simulink model "single_phase_afe_ttype"  (R2026b)
settings: Solver=ode23tb  StopTime=param.sim.simlength  FixedStep=param.sim.tc  MaxStep=param.glb_time.tc
values from neighbouring files (symbols this model uses):
  param = struct()    [init_model.m]
undefined symbols (not defined in the file or in its folder): magnitude
libraries: fl_lib x30, nesl_utility x22, single_phase_transformer_lib x3, phase_shift_filter_ccaller x2, lithium_ion_battery x1, dclink_for_three_levels x1, three_phase_voltage_with_frt_emulator x1, power_meter_iec x1, simulink x1, cstblocks_lti x1, single_phase_three_levels_PWM_modulator x1, moving_average_filter x1
(part 1 of 4)
settings Model: Creator=LTNBDA  LastModifiedBy=d.bagnara
settings SolverCC: AutoInsertRateTranBlk=on  SolverResetMethod=Robust  ZeroCrossAlgorithm=Adaptive  ZeroCrossControl=EnableAll
settings DataIOCC: DSMLogging=off  LimitDataPoints=on  MaxDataPoints=1  ReturnWorkspaceOutputs=off  SaveFormat=Array  SaveOutput=off  SaveTime=off  SignalLogging=off  SignalLoggingSaveFormat=ModelDataLogs
settings OptimizationCC: EfficientMapNaN2IntZero=off  LifeSpan=inf  MemsetInitFltsAndDblsToZero=off
settings DebuggingCC: ArithmeticOperatorsInVariantConditions=warning  FcnCallInpInsideContextMsg=warning  IgnoredZcDiagnostic=none  MergeDetectMultiDrivingBlocksExec=none  MultiTaskCondExecSysMsg=none  MultiTaskDSMMsg=warning  MultiTaskRateTransMsg=warning  SFNoUnconditionalDefaultTransitionDiag=warning  SFUnexpectedBacktrackingDiag=warning  SaveWithParameterizedLinksMsg=none  SignalResolutionControl=TryResolveAllWithWarning  SolverPrmCheckMsg=warning  StateNameClashWarn=warning  UnderspecifiedInitializationDetection=Classic
settings HardwareCC: ProdEndianess=Unspecified  ProdEqTarget=off  ProdHWDeviceType=Generic->64-bit Embedded Processor (LP64)  ProdIntDivRoundTo=Undefined  ProdLargestAtomicFloat=None  TargetEndianess=LittleEndian  TargetHWDeviceType=MATLAB Host  TargetIntDivRoundTo=Zero  TargetLongLongMode=on
settings ModelReferenceCC: PropagateSignalLabelsOutOfModel=off
settings SFSimCC: CustomCodeUndefinedFunction=UseInterfaceOnly  SimUseLocalCustomCode=off
settings SFSimCC: SimCustomHeaderCode=|
  | #include "rpi.h"
  | #include "rpi_simulink.h"
  | #include "mavgflt.h"
  | #include "mavgflt_simulink.h"
  | #include "mavgflts.h"
  | #include "mavgflts_simulink.h"
  | #include "dsmavgflt.h"
  | #include "dsmavgflt_simulink.h"
  | #include "bemf_obsv.h"
  | #include "bemf_obsv_simulink.h"
  | #include "bemf_obsv_load_est.h"
  | #include "bemf_obsv_load_est_simulink.h"
  | #include "dqvector_pi.h"
  | #include "dqvector_pi_simulink.h"
  | #include "sv_pwm_simulink.h"
  | #include "sv_pwm.h"
  | #include "first_harmonic_tracker.h"
  | #include "first_harmonic_tracker_simulink.h"
  | #include "dqpll_thyr.h"
  | #include "dqpll_thyr_simulink.h"
  | #include "dqpll_grid.h"
  | #include "dqpll_grid_simulink.h"
  | #include "phase_shift_flt_simulink.h"
  | #include "phase_shift_flt.h"
  | #include "sogi_flt_simulink.h"
  | #include "sogi_flt.h"
  | #include "linear_double_integrator_observer_simulink.h"
  | #include "linear_double_integrator_observer.h"
settings SFSimCC: SimUserIncludeDirs=|
  | include
  | src
settings SFSimCC: SimUserSources=|
  | "rpi.c"
  | "rpi_simulink.c"
  | "mavgflt_simulink.c"
  | "mavgflt.c"
  | "mavgflts_simulink.c"
  | "mavgflts.c"
  | "dsmavgflt_simulink.c"
  | "dsmavgflt.c"
  | "bemf_obsv_simulink.c"
  | "bemf_obsv.c"
  | "bemf_obsv_load_est_simulink.c"
  | "bemf_obsv_load_est.c"
  | "dqvector_pi.c"
  | "dqvector_pi_simulink.c"
  | "sv_pwm_simulink.c"
  | "sv_pwm.c"
  | "first_harmonic_tracker_simulink.c"
  | "first_harmonic_tracker.c"
  | "dqpll_thyr_simulink.c"
  | "dqpll_thyr.c"
  | "dqpll_grid_simulink.c"
  | "dqpll_grid.c"
  | "phase_shift_flt_simulink.c"
  | "phase_shift_flt.c"
  | "sogi_flt_simulink.c"
  | "sogi_flt.c"
  | "linear_double_integrator_observer_simulink.c"
  | "linear_double_integrator_observer.c"
settings RTWCC: RTWUseLocalCustomCode=off
settings CodeAppCC: StateflowObjectComments=on
settings GRTTargetCC: CombineOutputUpdateFcns=off  GRTInterface=on  TargetLangStandard=C89/C90 (ANSI)
settings ConfigComp: CovExternalEMLEnable=off  CovSaveCumulativeToWorkspaceVar=on  CovSaveSingleToWorkspaceVar=on
settings SimscapeCC: SimscapeNormalizeSystem=off  SimscapeUseEnergyAccounting=off

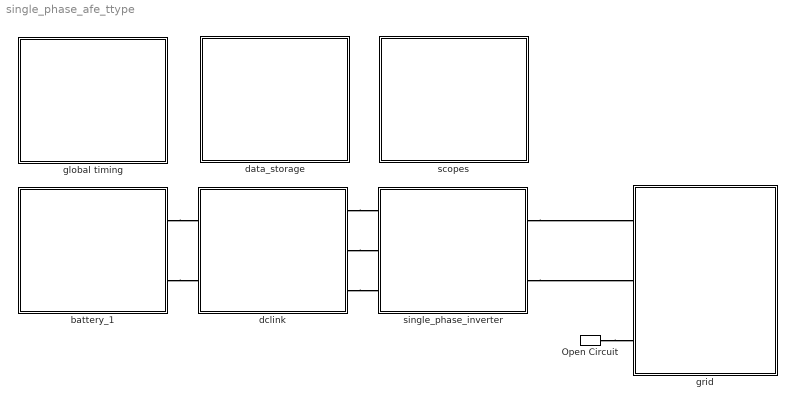
== system single_phase_afe_ttype ==
  Open Circuit : fl_lib/Electrical/Electrical Elements/Open Circuit  v_specify=off  v_priority=None  v=0 V  v_nominal_specify=off  v_nominal_value=1  v_nominal_unit=V
  battery_1 : Subsystem
  data_storage : Subsystem
  dclink : Subsystem
  global timing : Subsystem
  grid : Subsystem
  scopes : Subsystem
  single_phase_inverter : Subsystem
  connections:
  single_phase_inverter/RConn1 -- grid/RConn1
  single_phase_inverter/RConn2 -- grid/RConn2
  dclink/RConn1 -- single_phase_inverter/LConn1
  dclink/RConn2 -- single_phase_inverter/LConn2
  dclink/RConn3 -- single_phase_inverter/LConn3
  battery_1/RConn2 -- dclink/LConn2
  battery_1/RConn1 -- dclink/LConn1
  Open Circuit/LConn1 -- grid/RConn3

== system single_phase_afe_ttype/battery_1 ==
  To Workspace14 : ToWorkspace  VariableName=battery_1_data_sim  SampleTime=param.glb_time.tc
      settings: MaxDataPoints=param.glb_time.Nc  Decimation=param.glb_time.decimation_tc
  lithium ion battery : Scope
      settings: ActiveDisplayYMinimum=-1009.2320386548216  ActiveDisplayYMaximum=1611.8768779635091  DataLoggingVariableName=ScopeData3
  lithium_ion_battery : lithium_ion_battery/lithium_ion_battery  Q=param.battery.pack_1.Q  number_of_cells=param.battery.pack_1.number_of_cells  E_1=param.battery.pack_1.E_1  E0=param.battery.pack_1.E0  E1=param.battery.pack_1.E1  E2=param.battery.pack_1.E2  E3=param.battery.pack_1.E3  Elog=param.battery.pack_1.Elog  R0=param.battery.pack_1.R0  R1=param.battery.pack_1.R1  C1=param.battery.pack_1.C1  M=param.battery.pack_1.M  alpha=param.battery.pack_1.alpha  soc_init=param.battery.pack_1.soc_init  ts_battery=param.glb_time.ts_dab  q1Kalman=param.battery.pack_1.q1Kalman  q2Kalman=param.battery.pack_1.q2Kalman  q3Kalman=param.battery.pack_1.q3Kalman  rKalman=param.battery.pack_1.rKalman  tc=param.glb_time.tc  enable_white_noise_m=0  battery_voltage_init_m=param.battery.nominal_battery_voltage_1
  single_phase_ui_measure : Subsystem
  dc(+) : PMIOPort  Side=Right
  dc(-) : PMIOPort  Port=2  Side=Right
  wires:
  lithium_ion_battery/1 -> To Workspace14/1, lithium ion battery/1
  connections:
  single_phase_ui_measure/LConn2 -- lithium_ion_battery/RConn2
  single_phase_ui_measure/RConn1 -- dc(+)/RConn1
  single_phase_ui_measure/LConn1 -- lithium_ion_battery/RConn1
  dc(-)/RConn1 -- single_phase_ui_measure/RConn2

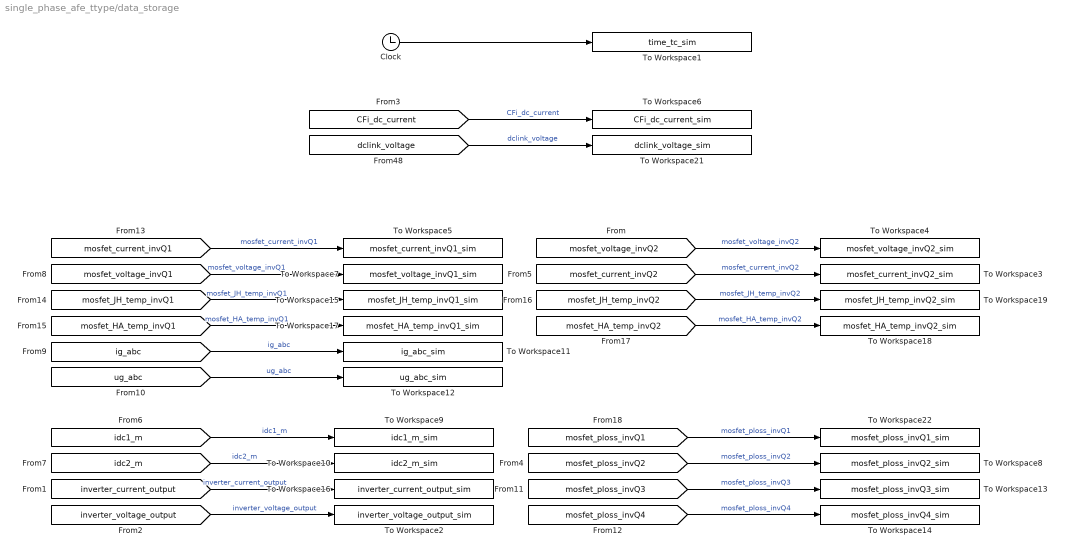
== system single_phase_afe_ttype/data_storage ==
  Clock : Clock
  To Workspace1 : ToWorkspace  VariableName=time_tc_sim  SampleTime=param.glb_time.tc
      settings: MaxDataPoints=param.glb_time.Nc  Decimation=param.glb_time.decimation_tc
  To Workspace10 : ToWorkspace  VariableName=idc2_m_sim  SampleTime=param.glb_time.tc
      settings: MaxDataPoints=param.glb_time.Nc  Decimation=param.glb_time.decimation_tc
  To Workspace11 : ToWorkspace  VariableName=ig_abc_sim  SampleTime=param.glb_time.tc
      settings: MaxDataPoints=param.glb_time.Nc  Decimation=param.glb_time.decimation_tc
  To Workspace12 : ToWorkspace  VariableName=ug_abc_sim  SampleTime=param.glb_time.tc
      settings: MaxDataPoints=param.glb_time.Nc  Decimation=param.glb_time.decimation_tc
  To Workspace13 : ToWorkspace  VariableName=mosfet_ploss_invQ3_sim  SampleTime=param.glb_time.tc
      settings: MaxDataPoints=param.glb_time.Nc  Decimation=param.glb_time.decimation_tc
  To Workspace14 : ToWorkspace  VariableName=mosfet_ploss_invQ4_sim  SampleTime=param.glb_time.tc
      settings: MaxDataPoints=param.glb_time.Nc  Decimation=param.glb_time.decimation_tc
  To Workspace15 : ToWorkspace  VariableName=mosfet_JH_temp_invQ1_sim  SampleTime=param.glb_time.tc
      settings: MaxDataPoints=param.glb_time.Nc  Decimation=param.glb_time.decimation_tc
  To Workspace16 : ToWorkspace  VariableName=inverter_current_output_sim  SampleTime=param.glb_time.tc
      settings: MaxDataPoints=param.glb_time.Nc  Decimation=param.glb_time.decimation_tc
  To Workspace17 : ToWorkspace  VariableName=mosfet_HA_temp_invQ1_sim  SampleTime=param.glb_time.tc
      settings: MaxDataPoints=param.glb_time.Nc  Decimation=param.glb_time.decimation_tc
  To Workspace18 : ToWorkspace  VariableName=mosfet_HA_temp_invQ2_sim  SampleTime=param.glb_time.tc
      settings: MaxDataPoints=param.glb_time.Nc  Decimation=param.glb_time.decimation_tc
  To Workspace19 : ToWorkspace  VariableName=mosfet_JH_temp_invQ2_sim  SampleTime=param.glb_time.tc
      settings: MaxDataPoints=param.glb_time.Nc  Decimation=param.glb_time.decimation_tc
  To Workspace2 : ToWorkspace  VariableName=inverter_voltage_output_sim  SampleTime=param.glb_time.tc
      settings: MaxDataPoints=param.glb_time.Nc  Decimation=param.glb_time.decimation_tc
  To Workspace21 : ToWorkspace  VariableName=dclink_voltage_sim  SampleTime=param.glb_time.tc
      settings: MaxDataPoints=param.glb_time.Nc  Decimation=param.glb_time.decimation_tc
  To Workspace22 : ToWorkspace  VariableName=mosfet_ploss_invQ1_sim  SampleTime=param.glb_time.tc
      settings: MaxDataPoints=param.glb_time.Nc  Decimation=param.glb_time.decimation_tc
  To Workspace3 : ToWorkspace  VariableName=mosfet_current_invQ2_sim  SampleTime=param.glb_time.tc
      settings: MaxDataPoints=param.glb_time.Nc  Decimation=param.glb_time.decimation_tc
  To Workspace4 : ToWorkspace  VariableName=mosfet_voltage_invQ2_sim  SampleTime=param.glb_time.tc
      settings: MaxDataPoints=param.glb_time.Nc  Decimation=param.glb_time.decimation_tc
  To Workspace5 : ToWorkspace  VariableName=mosfet_current_invQ1_sim  SampleTime=param.glb_time.tc
      settings: MaxDataPoints=param.glb_time.Nc  Decimation=param.glb_time.decimation_tc
  To Workspace6 : ToWorkspace  VariableName=CFi_dc_current_sim  SampleTime=param.glb_time.tc
      settings: MaxDataPoints=param.glb_time.Nc  Decimation=param.glb_time.decimation_tc
  To Workspace7 : ToWorkspace  VariableName=mosfet_voltage_invQ1_sim  SampleTime=param.glb_time.tc
      settings: MaxDataPoints=param.glb_time.Nc  Decimation=param.glb_time.decimation_tc
  To Workspace8 : ToWorkspace  VariableName=mosfet_ploss_invQ2_sim  SampleTime=param.glb_time.tc
      settings: MaxDataPoints=param.glb_time.Nc  Decimation=param.glb_time.decimation_tc
  To Workspace9 : ToWorkspace  VariableName=idc1_m_sim  SampleTime=param.glb_time.tc
      settings: MaxDataPoints=param.glb_time.Nc  Decimation=param.glb_time.decimation_tc
  wires:
  Clock/1 -> To Workspace1/1
  [inverter_current_output] -> To Workspace16/1  "inverter_current_output"
  [inverter_voltage_output] -> To Workspace2/1  "inverter_voltage_output"
  [CFi_dc_current] -> To Workspace6/1  "CFi_dc_current"
  [mosfet_ploss_invQ1] -> To Workspace22/1  "mosfet_ploss_invQ1"
  [dclink_voltage] -> To Workspace21/1  "dclink_voltage"
  [mosfet_current_invQ1] -> To Workspace5/1  "mosfet_current_invQ1"
  [mosfet_current_invQ2] -> To Workspace3/1  "mosfet_current_invQ2"
  [mosfet_voltage_invQ2] -> To Workspace4/1  "mosfet_voltage_invQ2"
  [mosfet_voltage_invQ1] -> To Workspace7/1  "mosfet_voltage_invQ1"
  [mosfet_ploss_invQ2] -> To Workspace8/1  "mosfet_ploss_invQ2"
  [ig_abc] -> To Workspace11/1  "ig_abc"
  [ug_abc] -> To Workspace12/1  "ug_abc"
  [mosfet_JH_temp_invQ1] -> To Workspace15/1  "mosfet_JH_temp_invQ1"
  [mosfet_HA_temp_invQ1] -> To Workspace17/1  "mosfet_HA_temp_invQ1"
  [mosfet_JH_temp_invQ2] -> To Workspace19/1  "mosfet_JH_temp_invQ2"
  [mosfet_HA_temp_invQ2] -> To Workspace18/1  "mosfet_HA_temp_invQ2"
  [idc1_m] -> To Workspace9/1  "idc1_m"
  [idc2_m] -> To Workspace10/1  "idc2_m"
  [mosfet_ploss_invQ4] -> To Workspace14/1  "mosfet_ploss_invQ4"
  [mosfet_ploss_invQ3] -> To Workspace13/1  "mosfet_ploss_invQ3"

== system single_phase_afe_ttype/dclink ==
  Open Circuit : fl_lib/Electrical/Electrical Elements/Open Circuit  v_specify=off  v_priority=None  v=0 V  v_nominal_specify=off  v_nominal_value=1  v_nominal_unit=V
  dclink : dclink_for_three_levels/dclink  Cdc1_m=param.afe.hw.CFi1  Cdc2_m=param.afe.hw.CFi2  Rudc_measure=param.afe.hw.Rudc_measure  Vdc_scale=param.afe.hw.udc_nom  Vdc1_m_init=param.afe.hw.udc1_init  Vdc2_m_init=param.afe.hw.udc2_init
  references : Subsystem
  Udc(+) : PMIOPort  Side=Right
  np : PMIOPort  Port=2  Side=Right
  Udc(-) : PMIOPort  Port=3  Side=Right
  udc(+) : PMIOPort  Port=4  Side=Left
  udc(-) : PMIOPort  Port=5  Side=Left
  wires:
  dclink/1 -> references/1(m)
  connections:
  Open Circuit/LConn1 -- dclink/RConn2
  udc(+)/RConn1 -- dclink/RConn1
  udc(-)/RConn1 -- dclink/RConn3
  Udc(+)/RConn1 -- dclink/LConn1
  Udc(-)/RConn1 -- dclink/LConn3
  dclink/LConn2 -- np/RConn1

== system single_phase_afe_ttype/global timing ==
  Unit Delay : UnitDelay  SampleTime=param.glb_time.tc
  time_afe1 : Subsystem  mask{k=1}
      mask prompts: k "Time Gain"
      mask Display:
      | disp('time-gen');
      | port_label('input', 1, 'crt');
      | port_label('output', 1, 'tout');
  time_afe3 : Subsystem  mask{k=1}
      mask prompts: k "Time Gain"
      mask Display:
      | disp('time-gen');
      | port_label('output', 1, 'tout');
  tag scope: master_time=global, time_inv_module_1=global
  wires:
  time_afe1/1(Out1) -> [time_inv_module_1]
  time_afe3/1(Out1) -> [master_time]
  [local_time_corr_llc_mod1] -> Unit Delay/1
  Unit Delay/1 -> time_afe1/1(correction_time)

== system single_phase_afe_ttype/grid ==
  Bus Selector : BusSelector  OutputSignals=Q1p,Q1n,P1n,P1p,U1n,U1p,i_act_1n,i_react_1n,i_act_1p,i_react_1p
  To Workspace1 : ToWorkspace  VariableName=i_react_1n  SampleTime=param.glb_time.ts_afe
      settings: MaxDataPoints=param.glb_time.Ns_afe
  To Workspace2 : ToWorkspace  VariableName=i_react_1p  SampleTime=param.glb_time.ts_afe
      settings: MaxDataPoints=param.glb_time.Ns_afe
  To Workspace3 : ToWorkspace  VariableName=i_act_1n  SampleTime=param.glb_time.ts_afe
      settings: MaxDataPoints=param.glb_time.Ns_afe
  To Workspace4 : ToWorkspace  VariableName=i_act_1p  SampleTime=param.glb_time.ts_afe
      settings: MaxDataPoints=param.glb_time.Ns_afe
  To Workspace5 : ToWorkspace  VariableName=u1p  SampleTime=param.glb_time.ts_afe
      settings: MaxDataPoints=param.glb_time.Ns_afe
  To Workspace6 : ToWorkspace  VariableName=u1n  SampleTime=param.glb_time.ts_afe
      settings: MaxDataPoints=param.glb_time.Ns_afe
  grid_emulator : Subsystem
  power meter iec1 : power_meter_iec/power meter iec  period=pi/param.grid.emu.omega_grid_nom  ts=param.glb_time.tc  enable_time=0.025
  threephase_vi_measures : Subsystem
  ua : PMIOPort  Side=Right
  ub : PMIOPort  Port=2  Side=Right
  uc : PMIOPort  Port=3  Side=Right
  tag scope: P1n_global=global, P1p_global=global, Q1n_global=global, Q1p_global=global
  wires:
  [gamma_grid_emulator] -> power meter iec1/1
  [ug_abc] -> power meter iec1/2
  [ig_abc] -> power meter iec1/3
  power meter iec1/1 -> Bus Selector/1
  Bus Selector/1 -> [Q1p_global]  "<Q1p>"
  Bus Selector/2 -> [Q1n_global]  "<Q1n>"
  Bus Selector/3 -> [P1n_global]  "<P1n>"
  Bus Selector/4 -> [P1p_global]  "<P1p>"
  Bus Selector/5 -> To Workspace6/1  "<U1n>"
  Bus Selector/6 -> To Workspace5/1  "<U1p>"
  Bus Selector/7 -> To Workspace3/1  "<i_act_1n>"
  Bus Selector/8 -> To Workspace1/1  "<i_react_1n>"
  Bus Selector/9 -> To Workspace4/1  "<i_act_1p>"
  Bus Selector/10 -> To Workspace2/1  "<i_react_1p>"
  [omega_grid_emulator] -> power meter iec1/4
  connections:
  threephase_vi_measures/LConn3 -- grid_emulator/RConn3
  threephase_vi_measures/LConn1 -- grid_emulator/RConn1
  threephase_vi_measures/RConn2 -- ub/RConn1
  threephase_vi_measures/LConn2 -- grid_emulator/RConn2
  threephase_vi_measures/RConn1 -- ua/RConn1
  threephase_vi_measures/RConn3 -- uc/RConn1

== system single_phase_afe_ttype/scopes ==
  Bus Creator : BusCreator  Inputs=2
  dclink voltage : Scope  NumInputPorts=3
      settings: SampleTime=param.glb_time.tc  ActiveDisplayString=3  ActiveDisplayYMinimum=-1788.34839052713  ActiveDisplayYMaximum=517.01346635999766  DataLoggingVariableName=ScopeData9
  ig_abc/ug_abc : Scope  NumInputPorts=2
      settings: SampleTime=param.glb_time.tc  ActiveDisplayYMinimum=-713.27946799108952  ActiveDisplayYMaximum=713.52801996826327  DataLoggingVariableName=ScopeData5
  input dc modA : Scope  NumInputPorts=2
      settings: SampleTime=param.glb_time.tc  ActiveDisplayYMinimum=-67.715483087935809  ActiveDisplayYMaximum=609.43655738592645  DataLoggingVariableName=ScopeData4
  inverter current/voltage : Scope  NumInputPorts=4
      settings: ActiveDisplayString=3  ActiveDisplayYMinimum=-1356.3487617019355  ActiveDisplayYMaximum=1011.5095624681422
  inverter current/voltage output : Scope  NumInputPorts=2
      settings: ActiveDisplayYMinimum=-809.40125502350236  ActiveDisplayYMaximum=818.72199299199281
  iu-mosfet-invQ1 : Scope  NumInputPorts=2
      settings: SampleTime=param.glb_time.tc  ActiveDisplayYMinimum=-1884.5917198054758  ActiveDisplayYMaximum=2532.7760155502147  DataLoggingVariableName=ScopeData7
  power_loss mosfet_inv : Scope  NumInputPorts=2
      settings: SampleTime=param.glb_time.tc  ActiveDisplayYMinimum=-70.3597503046535  ActiveDisplayYMaximum=633.23512274412  DataLoggingVariableName=ScopeData6
  wires:
  [idc1_m] -> inverter current/voltage/3  "idc1_m"
  [inverter_voltage_output] -> inverter current/voltage/2, inverter current/voltage output/1  "inverter_voltage_output_modA"
  [inverter_current_output] -> inverter current/voltage/1, inverter current/voltage output/2  "inverter_current_output_modA"
  [idc2_m] -> inverter current/voltage/4  "idc2_m"
  [idc1_m] -> input dc modA/1  "idc1_m"
  [idc2_m] -> input dc modA/2  "idc2_m"
  [ug_abc] -> ig_abc/ug_abc/2  "vg_abc"
  [ig_abc] -> ig_abc/ug_abc/1  "ig_abc"
  [mosfet_ploss_invQ1] -> power_loss mosfet_inv/1  "mosfet_ploss_invQ1"
  [mosfet_JH_temp_invQ1] -> Bus Creator/1  "mosfet_JH_temp_invQ1"
  [mosfet_HA_temp_invQ1] -> Bus Creator/2  "mosfet_HA_temp_invQ1"
  Bus Creator/1 -> power_loss mosfet_inv/2
  [mosfet_current_invQ1] -> iu-mosfet-invQ1/1  "mosfet_current_invQ1"
  [mosfet_voltage_invQ1] -> iu-mosfet-invQ1/2  "mosfet_voltage_invQ1"
  [dclink_voltage] -> dclink voltage/1  "dclink_voltage"
  [dclink_p2gnd_voltage] -> dclink voltage/2  "dclink_p2gnd_voltage"
  [dclink_n2gnd_voltage] -> dclink voltage/3  "dclink_n2gnd_voltage"

== system single_phase_afe_ttype/single_phase_inverter ==
  CFu : fl_lib/Electrical/Electrical Elements/Capacitor  c=param.afe.hw.CFu F  r=param.afe.hw.RCFu Ohm  g=0 1/Ohm  i_specify=off  i_priority=None  i=0 A  i_nominal_specify=off  i_nominal_value=1  i_nominal_unit=A  v_specify=off  v_priority=None  v=0 V  v_nominal_specify=off  v_nominal_value=1  v_nominal_unit=V  vc_specify=off  vc_priority=High  vc=0 V  vc_nominal_specify=off  vc_nominal_value=1  vc_nominal_unit=V
  LFu1 : fl_lib/Electrical/Electrical Elements/Inductor  l=param.afe.hw.LFu1 H  r=param.afe.hw.RLFu1 Ohm  g=1e-9 1/Ohm  i_specify=on  i_priority=High  i=0 A  i_nominal_specify=off  i_nominal_value=1  i_nominal_unit=A  v_specify=off  v_priority=None  v=0 V  v_nominal_specify=off  v_nominal_value=1  v_nominal_unit=V  i_L_specify=off  i_L_priority=High  i_L=0 A  i_L_nominal_specify=off  i_L_nominal_value=1  i_L_nominal_unit=A
  LFu2 : fl_lib/Electrical/Electrical Elements/Inductor  l=param.afe.hw.LFu2 H  r=param.afe.hw.RLFu2 Ohm  g=1e-9 1/Ohm  i_specify=on  i_priority=High  i=0 A  i_nominal_specify=off  i_nominal_value=1  i_nominal_unit=A  v_specify=off  v_priority=None  v=0 V  v_nominal_specify=off  v_nominal_value=1  v_nominal_unit=V  i_L_specify=off  i_L_priority=High  i_L=0 A  i_L_nominal_specify=off  i_L_nominal_value=1  i_L_nominal_unit=A
  single phase inverter control : Subsystem
  single_phase_inverter : Subsystem
  vi_measures_grid : Subsystem
  uac(+) : PMIOPort  Side=Right
  uac(-) : PMIOPort  Port=2  Side=Right
  udc(+) : PMIOPort  Port=3  Side=Left
  np : PMIOPort  Port=4  Side=Left
  udc(-) : PMIOPort  Port=5  Side=Left
  wires:
  single phase inverter control/1(gate_cmds) -> single_phase_inverter/1(gate_commands)
  connections:
  single_phase_inverter/LConn1 -- udc(+)/RConn1
  np/RConn1 -- single_phase_inverter/LConn2
  single_phase_inverter/LConn3 -- udc(-)/RConn1
  LFu1/RConn1 -- vi_measures_grid/RConn1 -- CFu/LConn1
  LFu2/RConn1 -- vi_measures_grid/RConn2 -- CFu/RConn1
  single_phase_inverter/RConn2 -- LFu2/LConn1
  single_phase_inverter/RConn1 -- LFu1/LConn1
  uac(+)/RConn1 -- vi_measures_grid/LConn1
  uac(-)/RConn1 -- vi_measures_grid/LConn2

== system single_phase_afe_ttype/battery_1/single_phase_ui_measure ==
  Bus Creator : BusCreator  Inputs=2
  Current Sensor : fl_lib/Electrical/Electrical Sensors/Current Sensor
  Selector : Selector  InputPortWidth=2  IndexOptions=Index vector (dialog)  Indices=2  OutputSizes=1  RuntimeRangeChecks=off
  Selector1 : Selector  InputPortWidth=2  IndexOptions=Index vector (dialog)  Indices=1  OutputSizes=1  RuntimeRangeChecks=off
  Voltage Sensor : fl_lib/Electrical/Electrical Sensors/Voltage Sensor
  dab input modA : Scope  NumInputPorts=2
      settings: SampleTime=param.glb_time.tc  ActiveDisplayYMinimum=-28.571537221503817  ActiveDisplayYMaximum=257.27265236106325  DataLoggingVariableName=ScopeData2
  iph : nesl_utility/PS-Simulink Converter  PhysicalDomain=network_engine_domain  SubClassName=ps_output  LeftPortType=input  RightPortType=output  PseudoPeriodic=off  Frequencies=[]  VectorFormat=1-D array  Unit=A  AffineConversion=off
  uph : nesl_utility/PS-Simulink Converter  PhysicalDomain=network_engine_domain  SubClassName=ps_output  LeftPortType=input  RightPortType=output  PseudoPeriodic=off  Frequencies=[]  VectorFormat=1-D array  Unit=V  AffineConversion=off
  Udc(+) : PMIOPort  Side=Left
  udc(+) : PMIOPort  Port=2  Side=Right
  Udc(-) : PMIOPort  Port=3  Side=Left
  udc(-) : PMIOPort  Port=4  Side=Right
  tag scope: current_battery_1=global, voltage_battery_1=global
  wires:
  Bus Creator/1 -> Selector/1, Selector1/1  "ui_data"
  iph/1 -> Bus Creator/1  "iph"
  uph/1 -> Bus Creator/2  "uph"
  Selector1/1 -> [current_battery_1], dab input modA/1  "current_battery"
  Selector/1 -> dab input modA/2, [voltage_battery_1]  "voltage_battery"
  connections:
  iph/LConn1 -- Current Sensor/RConn1
  Voltage Sensor/LConn1 -- Current Sensor/LConn1 -- Udc(+)/RConn1
  Current Sensor/RConn2 -- udc(+)/RConn1
  Voltage Sensor/RConn1 -- uph/LConn1
  Voltage Sensor/RConn2 -- Udc(-)/RConn1 -- udc(-)/RConn1

== system single_phase_afe_ttype/dclink/references ==
  m : Inport
  Bus Selector : BusSelector  OutputSignals=udc,udc_p_gnd,udc_n_gnd,Cdc1_current
  Bus Selector1 : BusSelector  OutputSignals=idc1,idc2
  tag scope: CFi_dc_current=global, dclink_n2gnd_voltage=global, dclink_p2gnd_voltage=global, dclink_voltage=global, idc1_m=global, idc2_m=global
  wires:
  m/1 -> Bus Selector/1, Bus Selector1/1
  Bus Selector1/1 -> [idc1_m]  "<idc1>"
  Bus Selector/1 -> [dclink_voltage]  "<udc>"
  Bus Selector/4 -> [CFi_dc_current]  "<Cdc1_current>"
  Bus Selector/3 -> [dclink_n2gnd_voltage]  "<udc_n_gnd>"
  Bus Selector/2 -> [dclink_p2gnd_voltage]  "<udc_p_gnd>"
  Bus Selector1/2 -> [idc2_m]  "<idc2>"

== system single_phase_afe_ttype/global timing/time_afe1 ==
  correction_time : Inport
  Constant : Constant
  Gain : Gain  Gain=k
  Product : Product
  Sum : Sum  Inputs=|++
  time_1 : Clock
  Out1 : Outport
  wires:
  time_1/1 -> Gain/1
  Gain/1 -> Product/1
  Product/1 -> Out1/1
  correction_time/1 -> Sum/1
  Sum/1 -> Product/2
  Constant/1 -> Sum/2

== system single_phase_afe_ttype/global timing/time_afe3 ==
  Gain : Gain  Gain=k
  time_1 : Clock
  Out1 : Outport
  wires:
  Gain/1 -> Out1/1
  time_1/1 -> Gain/1

== system single_phase_afe_ttype/grid/grid_emulator ==
  3ph_Dyg : Subsystem
  Bus Selector : BusSelector  OutputSignals=ua_grid_emu,ub_grid_emu,uc_grid_emu
  Bus Selector1 : BusSelector  OutputSignals=gamma_grid_emulator,omega_grid_emulator
  Controlled Voltage Source : fl_lib/Electrical/Electrical Sources/Controlled Voltage Source
  Controlled Voltage Source1 : fl_lib/Electrical/Electrical Sources/Controlled Voltage Source
  Controlled Voltage Source2 : fl_lib/Electrical/Electrical Sources/Controlled Voltage Source
  Electrical Reference : fl_lib/Electrical/Electrical Elements/Electrical Reference
  Simulink-PS Converter : nesl_utility/Simulink-PS Converter  PhysicalDomain=network_engine_domain  SubClassName=ps_input  LeftPortType=input  RightPortType=output  PseudoPeriodic=off  Frequencies=[]  NoiseDistribution=none  NoiseParameters=[]  Unit=V  AffineConversion=on  FilteringAndDerivatives=provide  SimscapeFilterOrder=1  InputFilterTimeConstant=0.001  UdotUserProvided=0
  Simulink-PS Converter1 : nesl_utility/Simulink-PS Converter  PhysicalDomain=network_engine_domain  SubClassName=ps_input  LeftPortType=input  RightPortType=output  PseudoPeriodic=off  Frequencies=[]  NoiseDistribution=none  NoiseParameters=[]  Unit=V  AffineConversion=on  FilteringAndDerivatives=provide  SimscapeFilterOrder=1  InputFilterTimeConstant=0.001  UdotUserProvided=0
  Simulink-PS Converter2 : nesl_utility/Simulink-PS Converter  PhysicalDomain=network_engine_domain  SubClassName=ps_input  LeftPortType=input  RightPortType=output  PseudoPeriodic=off  Frequencies=[]  NoiseDistribution=none  NoiseParameters=[]  Unit=V  AffineConversion=on  FilteringAndDerivatives=provide  SimscapeFilterOrder=1  InputFilterTimeConstant=0.001  UdotUserProvided=0
  Solver Configuration : nesl_utility/Solver Configuration  PhysicalDomain=network_engine_domain  SubClassName=solver  LeftPortType=input  RightPortType=generic  Tones=[]  Harmonics=[]  SimulateNoise=off  Profile=off  UseLocalSampling=off  EnableSwitchedLinearOptims=on  FrequencyDomain=off  UseCCode=off  RelTol=0.001  AbsTol=0.001  MinStep=1e-09  ToWorkspace=off  RevertToSquareIcSolve=off  NumHomotopyIterations=100  PhasorMode=off  PhasorModeNumHarmonics=1  ConsistencySolver=NEWTON_FTOL  CanonicalOrdering=UNORDERED  OptimizeIntermediates=UNOPTIMIZED  MulticoreSolverChoice=BACKWARD_EULER  IndexReductionMethod=DerivativeReplacement  DoDC=on  ResidualTolerance=1e-09  ConsistencyTolSource=GLOBAL  ConsistencyAbsTol=0.001  ConsistencyRelTol=0.001  ConsistencyTolFactor=0.001  UseLocalSolver=on  LocalSolverChoice=NE_BACKWARD_EULER_ADVANCER  ResolveIndetEquations=on  FunctionEvalNumThread=1  LocalSolverSampleTime=param.glb_time.tc  DoFixedCost=on  MaxNonlinIter=param.sim.nonlinear_iterations  MaxModeIter=2  ComputeImpulses=off  ImpulseIterations=2  LinearAlgebra=auto  LinearAlgebraNumThread=0  EquationFormulation=NE_TIME_EF  DelaysMemoryBudget=1024  AutomaticFiltering=on  FilteringTimeConstant=0.001  PartitionStorageMethod=AS_NEEDED  PartitionMemoryBudget=1024  PartitionMethod=BALANCED  MultibodyUseLocalSolver=off  MultibodyLocalSolverChoice=ODE1  MultibodyLocalSolverSampleTime=0.001
  three_phase_voltage_source_with_frt_emulator : three_phase_voltage_with_frt_emulator/three_phase_voltage_source_with_frt_emulator  nominal_frequency_m=param.grid.emu.fgrid_nom  nominal_voltage_m=param.grid.emu.us_nom  Vemu_ref_norm_m=param.grid.emu.Vemu_ref_norm  vp_xi_pu_m=param.grid.emu.up_xi_pu_ref  vp_eta_pu_m=param.grid.emu.up_eta_pu_ref  vn_xi_pu_m=param.grid.emu.un_xi_pu_ref  vn_eta_pu_m=param.grid.emu.un_eta_pu_ref  Am=param.grid.emu.sof_50Hz.A  Bm=param.grid.emu.sof_50Hz.B  Cm=param.grid.emu.sof_50Hz.C  enable_frt_1_m=param.grid.frt.enable_frt_1  enable_frt_2_m=param.grid.frt.enable_frt_2  start_time_LVRT_m=param.grid.frt.start_time_LVRT  end_time_LVRT_m=param.grid.frt.end_time_LVRT  deepPOSxi_m=param.grid.frt.deepPOSxi  deepPOSeta_m=param.grid.frt.deepPOSeta  deepNEGxi_m=param.grid.frt.deepNEGxi  deepNEGeta_m=param.grid.frt.deepNEGeta  Amplitude_U_m=param.grid.frt.Amplitude_U  Amplitude_V_m=param.grid.frt.Amplitude_V  Amplitude_W_m=param.grid.frt.Amplitude_W  t_ramp_m=param.grid.frt.t_ramp  Phase_shift_m=param.grid.frt.Phase_shift
  threephase_vi_measures : Subsystem
  u1 : PMIOPort  Side=Right
  u2 : PMIOPort  Port=2  Side=Right
  u3 : PMIOPort  Port=3  Side=Right
  tag scope: gamma_grid_emulator=global, omega_grid_emulator=global
  wires:
  Bus Selector1/2 -> [omega_grid_emulator]  "<omega_grid_emulator>"
  Bus Selector1/1 -> [gamma_grid_emulator]  "<gamma_grid_emulator>"
  Bus Selector/2 -> Simulink-PS Converter1/1  "<ub_grid_emu>"
  Bus Selector/3 -> Simulink-PS Converter2/1  "<uc_grid_emu>"
  three_phase_voltage_source_with_frt_emulator/1 -> Bus Selector1/1, Bus Selector/1
  Bus Selector/1 -> Simulink-PS Converter/1  "<ua_grid_emu>"
  connections:
  Simulink-PS Converter/RConn1 -- Controlled Voltage Source/RConn1
  Simulink-PS Converter1/RConn1 -- Controlled Voltage Source1/RConn1
  Simulink-PS Converter2/RConn1 -- Controlled Voltage Source2/RConn1
  Electrical Reference/LConn1 -- Controlled Voltage Source/RConn2 -- Controlled Voltage Source1/RConn2 -- Controlled Voltage Source2/RConn2 -- Solver Configuration/RConn1
  3ph_Dyg/RConn1 -- u1/RConn1
  3ph_Dyg/RConn2 -- u2/RConn1
  3ph_Dyg/RConn3 -- u3/RConn1
  3ph_Dyg/LConn1 -- threephase_vi_measures/RConn1
  3ph_Dyg/LConn2 -- threephase_vi_measures/RConn2
  3ph_Dyg/LConn3 -- threephase_vi_measures/RConn3
  Controlled Voltage Source/LConn1 -- threephase_vi_measures/LConn1
  Controlled Voltage Source1/LConn1 -- threephase_vi_measures/LConn2
  Controlled Voltage Source2/LConn1 -- threephase_vi_measures/LConn3

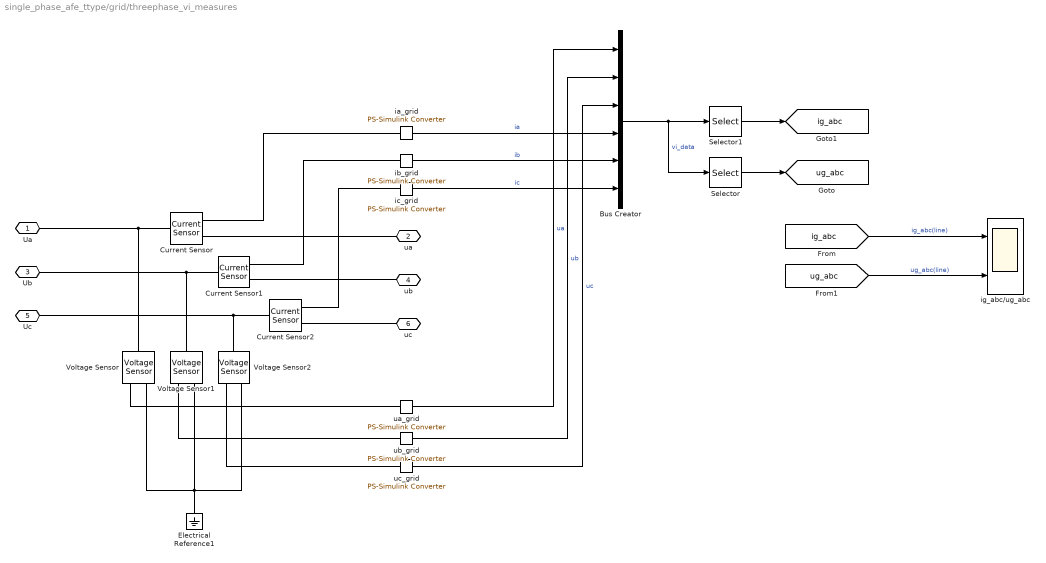
== system single_phase_afe_ttype/grid/threephase_vi_measures ==
  Bus Creator : BusCreator  Inputs=6
  Current Sensor : fl_lib/Electrical/Electrical Sensors/Current Sensor
  Current Sensor1 : fl_lib/Electrical/Electrical Sensors/Current Sensor
  Current Sensor2 : fl_lib/Electrical/Electrical Sensors/Current Sensor
  Electrical Reference1 : fl_lib/Electrical/Electrical Elements/Electrical Reference
  Selector : Selector  InputPortWidth=6  IndexOptions=Index vector (dialog)  Indices=[1 2 3]  OutputSizes=1  RuntimeRangeChecks=off
  Selector1 : Selector  InputPortWidth=6  IndexOptions=Index vector (dialog)  Indices=[4 5 6]  OutputSizes=1  RuntimeRangeChecks=off
  Voltage Sensor : fl_lib/Electrical/Electrical Sensors/Voltage Sensor
  Voltage Sensor1 : fl_lib/Electrical/Electrical Sensors/Voltage Sensor
  Voltage Sensor2 : fl_lib/Electrical/Electrical Sensors/Voltage Sensor
  ia_grid : nesl_utility/PS-Simulink Converter  PhysicalDomain=network_engine_domain  SubClassName=ps_output  LeftPortType=input  RightPortType=output  PseudoPeriodic=off  Frequencies=[]  VectorFormat=1-D array  Unit=A  AffineConversion=off
  ib_grid : nesl_utility/PS-Simulink Converter  PhysicalDomain=network_engine_domain  SubClassName=ps_output  LeftPortType=input  RightPortType=output  PseudoPeriodic=off  Frequencies=[]  VectorFormat=1-D array  Unit=A  AffineConversion=off
  ic_grid : nesl_utility/PS-Simulink Converter  PhysicalDomain=network_engine_domain  SubClassName=ps_output  LeftPortType=input  RightPortType=output  PseudoPeriodic=off  Frequencies=[]  VectorFormat=1-D array  Unit=A  AffineConversion=off
  ig_abc/ug_abc : Scope  NumInputPorts=2
      settings: SampleTime=param.glb_time.tc  ActiveDisplayYMinimum=-662.618491750231  ActiveDisplayYMaximum=662.00821995187164  DataLoggingVariableName=ScopeData2
  ua_grid : nesl_utility/PS-Simulink Converter  PhysicalDomain=network_engine_domain  SubClassName=ps_output  LeftPortType=input  RightPortType=output  PseudoPeriodic=off  Frequencies=[]  VectorFormat=1-D array  Unit=V  AffineConversion=off
  ub_grid : nesl_utility/PS-Simulink Converter  PhysicalDomain=network_engine_domain  SubClassName=ps_output  LeftPortType=input  RightPortType=output  PseudoPeriodic=off  Frequencies=[]  VectorFormat=1-D array  Unit=V  AffineConversion=off
  uc_grid : nesl_utility/PS-Simulink Converter  PhysicalDomain=network_engine_domain  SubClassName=ps_output  LeftPortType=input  RightPortType=output  PseudoPeriodic=off  Frequencies=[]  VectorFormat=1-D array  Unit=V  AffineConversion=off
  Ua : PMIOPort  Side=Left
  ua : PMIOPort  Port=2  Side=Right
  Ub : PMIOPort  Port=3  Side=Left
  ub : PMIOPort  Port=4  Side=Right
  Uc : PMIOPort  Port=5  Side=Left
  uc : PMIOPort  Port=6  Side=Right
  tag scope: ig_abc=global, ug_abc=global
  wires:
  Bus Creator/1 -> Selector1/1, Selector/1  "vi_data"
  Selector/1 -> [ug_abc]
  ib_grid/1 -> Bus Creator/5  "ib"
  ia_grid/1 -> Bus Creator/4  "ia"
  ic_grid/1 -> Bus Creator/6  "ic"
  ua_grid/1 -> Bus Creator/1  "ua"
  ub_grid/1 -> Bus Creator/2  "ub"
  uc_grid/1 -> Bus Creator/3  "uc"
  Selector1/1 -> [ig_abc]
  [ug_abc] -> ig_abc/ug_abc/2  "ug_abc(line)"
  [ig_abc] -> ig_abc/ug_abc/1  "ig_abc(line)"
  connections:
  Current Sensor1/LConn1 -- Ub/RConn1 -- Voltage Sensor1/LConn1
  Electrical Reference1/LConn1 -- Voltage Sensor/RConn2 -- Voltage Sensor2/RConn2 -- Voltage Sensor1/RConn2
  Voltage Sensor/RConn1 -- ua_grid/LConn1
  Current Sensor/RConn2 -- ua/RConn1
  Voltage Sensor1/RConn1 -- ub_grid/LConn1
  Voltage Sensor2/LConn1 -- Current Sensor2/LConn1 -- Uc/RConn1
  Current Sensor/LConn1 -- Ua/RConn1 -- Voltage Sensor/LConn1
  Current Sensor1/RConn2 -- ub/RConn1
  Voltage Sensor2/RConn1 -- uc_grid/LConn1
  ib_grid/LConn1 -- Current Sensor1/RConn1
  ia_grid/LConn1 -- Current Sensor/RConn1
  ic_grid/LConn1 -- Current Sensor2/RConn1
  Current Sensor2/RConn2 -- uc/RConn1

== system single_phase_afe_ttype/single_phase_inverter/single phase inverter control ==
  acquisition_and_scaling_current : Subsystem  Commented=on
  acquisition_and_scaling_current_with_white_noise : Subsystem
  acquisition_and_scaling_dc_voltage : Subsystem
  acquisition_and_scaling_grid_voltage_ac : Subsystem
  acquisition_and_scaling_voltage : Subsystem
  inverter_current_output_pu_reference : Subsystem
  pwm modulator : Subsystem
  single_phase_inverter_ctrl : Subsystem
  gate_cmds : Outport
  wires:
  [inverter_current_output] -> acquisition_and_scaling_current_with_white_noise/1(in)
  pwm modulator/1(gate_cmds) -> gate_cmds/1
  [TRGO_INV_1] -> single_phase_inverter_ctrl/Trigger
  [inverter_voltage_output] -> acquisition_and_scaling_voltage/1(in)
  single_phase_inverter_ctrl/1(u_ctrl_out) -> pwm modulator/1(vout)
  acquisition_and_scaling_current_with_white_noise/1(out) -> single_phase_inverter_ctrl/2(inverter_current_output_pu)  "inverter_current_output_pu"
  acquisition_and_scaling_voltage/1(out) -> single_phase_inverter_ctrl/1(inverter_voltage_output_pu)  "inverter_voltage_output_pu"
  inverter_current_output_pu_reference/1(inverter_current_output_pu_reference) -> single_phase_inverter_ctrl/3(inverter_current output_pu_reference)  "inverter_current_output_pu_reference"
  [dclink_voltage] -> acquisition_and_scaling_dc_voltage/1(in)
  acquisition_and_scaling_dc_voltage/1(out) -> single_phase_inverter_ctrl/4(dclink_voltage_pu)  "dclink_voltage_pu"
  [time_inv_module_1] -> single_phase_inverter_ctrl/5(local_time)
  [ug_abc] -> acquisition_and_scaling_grid_voltage_ac/1(in)
  acquisition_and_scaling_grid_voltage_ac/1(out) -> single_phase_inverter_ctrl/6(ugrid_pu)  "ug_abc"

== system single_phase_afe_ttype/single_phase_inverter/single_phase_inverter ==
  gate_commands : Inport
  Current Sensor : fl_lib/Electrical/Electrical Sensors/Current Sensor
  Voltage Sensor1 : fl_lib/Electrical/Electrical Sensors/Voltage Sensor
  iph : nesl_utility/PS-Simulink Converter  PhysicalDomain=network_engine_domain  SubClassName=ps_output  LeftPortType=input  RightPortType=output  PseudoPeriodic=off  Frequencies=[]  VectorFormat=1-D array  Unit=A  AffineConversion=off
  single phase inverter : Subsystem
      settings: PortSchema="{\"entries\":[{\"content\":{\"sides\":[{\"content\":{\"connectorIds\":[\"LConn1\",\"LConn2\"]},\"type\":\"ConnectorPlacement.EquallySpacedRectSide\",\"uuid\":\"4fcf4fea-d38f-431b-8a91-be3ce9782faf\"},{\"content\":{\"connectorIds\":[\"RConn1\",\"RConn2\",\"RConn3\"],\"side\":\"RIGHT\"},\"type\":\"ConnectorPlacement.EquallySpacedRectSide\",\"uuid\":\"0aa56277-92e9-4e3b-84c7-43398254a4d8\"},{\"content\":{\"connectorIds\":[\"In1\"],\"side\":\"TOP\"},\"type\":\"ConnectorPlacement.EquallySpacedRectSide\",\"uuid\":\"5cd150dc-bcaf-4cd7-b2a8-3db203726730\"}]},\"type\":\"ConnectorPlacement.EquallySpacedConnector\",\"uuid\":\"bf8194c4-c327-4d40-bea4-f1e7617f80b4\"}],\"packageUris\":[\"http://schema.mathworks.com/mf0/Connector/R2020b\"],\"version\":\"1.0\"}"
  uph1 : nesl_utility/PS-Simulink Converter  PhysicalDomain=network_engine_domain  SubClassName=ps_output  LeftPortType=input  RightPortType=output  PseudoPeriodic=off  Frequencies=[]  VectorFormat=1-D array  Unit=V  AffineConversion=off
  uac(+) : PMIOPort  Side=Right
  uac(-) : PMIOPort  Port=2  Side=Right
  udc(+) : PMIOPort  Port=3  Side=Left
  np : PMIOPort  Port=4  Side=Left
  udc(-) : PMIOPort  Port=5  Side=Left
  tag scope: inverter_current_output=global, inverter_voltage_output=global
  wires:
  iph/1 -> [inverter_current_output]  "inverter_current_output"
  uph1/1 -> [inverter_voltage_output]  "inverter_voltage_output"
  gate_commands/1 -> single phase inverter/1(gate_commands)
  connections:
  Current Sensor/RConn2 -- uac(+)/RConn1 -- Voltage Sensor1/LConn1
  single phase inverter/RConn1 -- udc(+)/RConn1
  iph/LConn1 -- Current Sensor/RConn1
  np/RConn1 -- single phase inverter/RConn2
  single phase inverter/LConn2 -- uac(-)/RConn1 -- Voltage Sensor1/RConn2
  Voltage Sensor1/RConn1 -- uph1/LConn1
  single phase inverter/LConn1 -- Current Sensor/LConn1
  single phase inverter/RConn3 -- udc(-)/RConn1

== system single_phase_afe_ttype/single_phase_inverter/vi_measures_grid ==
  Current Sensor : fl_lib/Electrical/Electrical Sensors/Current Sensor
  Gain1 : Gain  Gain=1/param.meas.ugrid_bez
  Gain6 : Gain  Gain=1/param.meas.igrid_bez
  Voltage Sensor : fl_lib/Electrical/Electrical Sensors/Voltage Sensor
  ia_grid : nesl_utility/PS-Simulink Converter  PhysicalDomain=network_engine_domain  SubClassName=ps_output  LeftPortType=input  RightPortType=output  PseudoPeriodic=off  Frequencies=[]  VectorFormat=1-D array  Unit=A  AffineConversion=off
  ua_grid : nesl_utility/PS-Simulink Converter  PhysicalDomain=network_engine_domain  SubClassName=ps_output  LeftPortType=input  RightPortType=output  PseudoPeriodic=off  Frequencies=[]  VectorFormat=1-D array  Unit=V  AffineConversion=off
  Ua : PMIOPort  Side=Left
  ua : PMIOPort  Port=2  Side=Right
  Ub : PMIOPort  Port=3  Side=Left
  ub : PMIOPort  Port=4  Side=Right
  tag scope: ig_pu_mod1=global, ug_pu_mod1=global
  wires:
  ua_grid/1 -> Gain1/1
  ia_grid/1 -> Gain6/1
  Gain1/1 -> [ug_pu_mod1]  "ua_grid_pu"
  Gain6/1 -> [ig_pu_mod1]  "ia_grid_pu"
  connections:
  ia_grid/LConn1 -- Current Sensor/RConn1
  Voltage Sensor/LConn1 -- Current Sensor/LConn1 -- Ua/RConn1
  Current Sensor/RConn2 -- ua/RConn1
  Voltage Sensor/RConn1 -- ua_grid/LConn1
  Voltage Sensor/RConn2 -- ub/RConn1 -- Ub/RConn1

== system single_phase_afe_ttype/grid/grid_emulator/3ph_Dyg ==
  Electrical Reference1 : fl_lib/Electrical/Electrical Elements/Electrical Reference
  ph1 : single_phase_transformer_lib/single phase transformer  Lm=param.grid.emu.trafo.Lm1 H  n1=param.grid.emu.trafo.n1  n2=param.grid.emu.trafo.n2  Rd1=param.grid.emu.trafo.Rd1 Ohm  Rd2=param.grid.emu.trafo.Rd2 Ohm  Ld1=param.grid.emu.trafo.Ld1 H  Ld2=param.grid.emu.trafo.Ld2 H  Rfe=param.grid.emu.trafo.Rfe1 Ohm  phi_specify=off  phi_priority=None  phi=0 V*s  phi_nominal_specify=off  phi_nominal_value=1  phi_nominal_unit=V*s  i1_specify=off  i1_priority=None  i1=0 A  i1_nominal_specify=off  i1_nominal_value=1  i1_nominal_unit=A  i2_specify=off  i2_priority=None  i2=0 A  i2_nominal_specify=off  i2_nominal_value=1  i2_nominal_unit=A  ife_specify=off  ife_priority=None  ife=0 A  ife_nominal_specify=off  ife_nominal_value=1  ife_nominal_unit=A  u1_specify=off  u1_priority=None  u1=0 V  u1_nominal_specify=off  u1_nominal_value=1  u1_nominal_unit=V  u2_specify=off  u2_priority=None  u2=0 V  u2_nominal_specify=off  u2_nominal_value=1  u2_nominal_unit=V
  ph2 : single_phase_transformer_lib/single phase transformer  Lm=param.grid.emu.trafo.Lm1 H  n1=param.grid.emu.trafo.n1  n2=param.grid.emu.trafo.n2  Rd1=param.grid.emu.trafo.Rd1 Ohm  Rd2=param.grid.emu.trafo.Rd2 Ohm  Ld1=param.grid.emu.trafo.Ld1 H  Ld2=param.grid.emu.trafo.Ld2 H  Rfe=param.grid.emu.trafo.Rfe1 Ohm  phi_specify=off  phi_priority=None  phi=0 V*s  phi_nominal_specify=off  phi_nominal_value=1  phi_nominal_unit=V*s  i1_specify=off  i1_priority=None  i1=0 A  i1_nominal_specify=off  i1_nominal_value=1  i1_nominal_unit=A  i2_specify=off  i2_priority=None  i2=0 A  i2_nominal_specify=off  i2_nominal_value=1  i2_nominal_unit=A  ife_specify=off  ife_priority=None  ife=0 A  ife_nominal_specify=off  ife_nominal_value=1  ife_nominal_unit=A  u1_specify=off  u1_priority=None  u1=0 V  u1_nominal_specify=off  u1_nominal_value=1  u1_nominal_unit=V  u2_specify=off  u2_priority=None  u2=0 V  u2_nominal_specify=off  u2_nominal_value=1  u2_nominal_unit=V
  ph3 : single_phase_transformer_lib/single phase transformer  Lm=param.grid.emu.trafo.Lm1 H  n1=param.grid.emu.trafo.n1  n2=param.grid.emu.trafo.n2  Rd1=param.grid.emu.trafo.Rd1 Ohm  Rd2=param.grid.emu.trafo.Rd2 Ohm  Ld1=param.grid.emu.trafo.Ld1 H  Ld2=param.grid.emu.trafo.Ld2 H  Rfe=param.grid.emu.trafo.Rfe1 Ohm  phi_specify=off  phi_priority=None  phi=0 V*s  phi_nominal_specify=off  phi_nominal_value=1  phi_nominal_unit=V*s  i1_specify=off  i1_priority=None  i1=0 A  i1_nominal_specify=off  i1_nominal_value=1  i1_nominal_unit=A  i2_specify=off  i2_priority=None  i2=0 A  i2_nominal_specify=off  i2_nominal_value=1  i2_nominal_unit=A  ife_specify=off  ife_priority=None  ife=0 A  ife_nominal_specify=off  ife_nominal_value=1  ife_nominal_unit=A  u1_specify=off  u1_priority=None  u1=0 V  u1_nominal_specify=off  u1_nominal_value=1  u1_nominal_unit=V  u2_specify=off  u2_priority=None  u2=0 V  u2_nominal_specify=off  u2_nominal_value=1  u2_nominal_unit=V
  ua : PMIOPort  Side=Right
  ub : PMIOPort  Port=2  Side=Right
  uc : PMIOPort  Port=3  Side=Right
  Ua : PMIOPort  Port=4  Side=Left
  Ub : PMIOPort  Port=5  Side=Left
  Uc : PMIOPort  Port=6  Side=Left
  connections:
  Electrical Reference1/LConn1 -- ph3/RConn2 -- ph2/RConn2 -- ph1/RConn2
  ph3/RConn1 -- uc/RConn1
  ph1/LConn1 -- ph3/LConn2 -- Ua/RConn1
  ph1/RConn1 -- ua/RConn1
  ph2/RConn1 -- ub/RConn1
  ph1/LConn2 -- ph2/LConn1 -- Ub/RConn1
  Uc/RConn1 -- ph3/LConn1 -- ph2/LConn2

== system single_phase_afe_ttype/grid/grid_emulator/threephase_vi_measures ==
  Bus Creator : BusCreator  Inputs=6
  Current Sensor : fl_lib/Electrical/Electrical Sensors/Current Sensor
  Current Sensor1 : fl_lib/Electrical/Electrical Sensors/Current Sensor
  Current Sensor2 : fl_lib/Electrical/Electrical Sensors/Current Sensor
  Electrical Reference1 : fl_lib/Electrical/Electrical Elements/Electrical Reference
  Voltage Sensor : fl_lib/Electrical/Electrical Sensors/Voltage Sensor
  Voltage Sensor1 : fl_lib/Electrical/Electrical Sensors/Voltage Sensor
  Voltage Sensor2 : fl_lib/Electrical/Electrical Sensors/Voltage Sensor
  i : Selector  InputPortWidth=6  IndexOptions=Index vector (dialog)  Indices=[4 5 6]  OutputSizes=1  RuntimeRangeChecks=off
  ia_grid : nesl_utility/PS-Simulink Converter  PhysicalDomain=network_engine_domain  SubClassName=ps_output  LeftPortType=input  RightPortType=output  PseudoPeriodic=off  Frequencies=[]  VectorFormat=1-D array  Unit=A  AffineConversion=off
  ib_grid : nesl_utility/PS-Simulink Converter  PhysicalDomain=network_engine_domain  SubClassName=ps_output  LeftPortType=input  RightPortType=output  PseudoPeriodic=off  Frequencies=[]  VectorFormat=1-D array  Unit=A  AffineConversion=off
  ic_grid : nesl_utility/PS-Simulink Converter  PhysicalDomain=network_engine_domain  SubClassName=ps_output  LeftPortType=input  RightPortType=output  PseudoPeriodic=off  Frequencies=[]  VectorFormat=1-D array  Unit=A  AffineConversion=off
  u : Selector  InputPortWidth=6  IndexOptions=Index vector (dialog)  Indices=[1 2 3]  OutputSizes=1  RuntimeRangeChecks=off
  ua_grid : nesl_utility/PS-Simulink Converter  PhysicalDomain=network_engine_domain  SubClassName=ps_output  LeftPortType=input  RightPortType=output  PseudoPeriodic=off  Frequencies=[]  VectorFormat=1-D array  Unit=V  AffineConversion=off
  ub_grid : nesl_utility/PS-Simulink Converter  PhysicalDomain=network_engine_domain  SubClassName=ps_output  LeftPortType=input  RightPortType=output  PseudoPeriodic=off  Frequencies=[]  VectorFormat=1-D array  Unit=V  AffineConversion=off
  uc_grid : nesl_utility/PS-Simulink Converter  PhysicalDomain=network_engine_domain  SubClassName=ps_output  LeftPortType=input  RightPortType=output  PseudoPeriodic=off  Frequencies=[]  VectorFormat=1-D array  Unit=V  AffineConversion=off
  Ua : PMIOPort  Side=Left
  ua : PMIOPort  Port=2  Side=Right
  Ub : PMIOPort  Port=3  Side=Left
  ub : PMIOPort  Port=4  Side=Right
  Uc : PMIOPort  Port=5  Side=Left
  uc : PMIOPort  Port=6  Side=Right
  tag scope: i_abc_line=global, u_abc_line=global
  wires:
  Bus Creator/1 -> i/1, u/1  "vi_data"
  ib_grid/1 -> Bus Creator/5  "ib"
  ia_grid/1 -> Bus Creator/4  "ia"
  ic_grid/1 -> Bus Creator/6  "ic"
  ua_grid/1 -> Bus Creator/1  "ua"
  ub_grid/1 -> Bus Creator/2  "ub"
  uc_grid/1 -> Bus Creator/3  "uc"
  i/1 -> [i_abc_line]
  u/1 -> [u_abc_line]
  connections:
  Current Sensor1/LConn1 -- Ub/RConn1 -- Voltage Sensor1/LConn1
  Electrical Reference1/LConn1 -- Voltage Sensor/RConn2 -- Voltage Sensor2/RConn2 -- Voltage Sensor1/RConn2
  Voltage Sensor/RConn1 -- ua_grid/LConn1
  Current Sensor/RConn2 -- ua/RConn1
  Voltage Sensor1/RConn1 -- ub_grid/LConn1
  Voltage Sensor2/LConn1 -- Current Sensor2/LConn1 -- Uc/RConn1
  Current Sensor/LConn1 -- Ua/RConn1 -- Voltage Sensor/LConn1
  Current Sensor1/RConn2 -- ub/RConn1
  Voltage Sensor2/RConn1 -- uc_grid/LConn1
  ib_grid/LConn1 -- Current Sensor1/RConn1
  ia_grid/LConn1 -- Current Sensor/RConn1
  ic_grid/LConn1 -- Current Sensor2/RConn1
  Current Sensor2/RConn2 -- uc/RConn1

== system single_phase_afe_ttype/single_phase_inverter/single phase inverter control/acquisition_and_scaling_current ==
  in : Inport
  1/Ti5 : Gain  Gain=1/param.afe.hw.ibez  SaturateOnIntegerOverflow=on  OutDataTypeStr=Inherit: Same as input  ParamDataTypeStr=Inherit: Same as input
  Quantizer : Quantizer  QuantizationInterval=param.meas.adc_quantization
  out : Outport
  wires:
  Quantizer/1 -> out/1
  1/Ti5/1 -> Quantizer/1
  in/1 -> 1/Ti5/1

== system single_phase_afe_ttype/single_phase_inverter/single phase inverter control/acquisition_and_scaling_current_with_white_noise ==
  in : Inport
  1/Ti5 : Gain  Gain=1/param.afe.hw.ibez  SaturateOnIntegerOverflow=on  OutDataTypeStr=Inherit: Same as input  ParamDataTypeStr=Inherit: Same as input
  Band-Limited White Noise : simulink/Sources/Band-Limited White Noise  Commented=on  Cov=1e-10  Ts=param.glb_time.tc  seed=[23341]
  Quantizer : Quantizer  QuantizationInterval=param.meas.adc_quantization
  Sum : Sum  Inputs=|++
  current_measure_with-without noise : Scope  NumInputPorts=2
      settings: ActiveDisplayYMinimum=-1.259685411609524  ActiveDisplayYMaximum=1.2603394332468927  DataLoggingVariableName=ScopeData15
  out : Outport
  wires:
  in/1 -> 1/Ti5/1
  1/Ti5/1 -> Sum/1, current_measure_with-without noise/1  "iload_without_noise"
  Sum/1 -> Quantizer/1
  Band-Limited White Noise/1 -> Sum/2
  Quantizer/1 -> out/1, current_measure_with-without noise/2  "iload_with_noise"

== system single_phase_afe_ttype/single_phase_inverter/single phase inverter control/acquisition_and_scaling_dc_voltage ==
  in : Inport
  1/Ti3 : Gain  Gain=1/param.afe.hw.udc_nom  SaturateOnIntegerOverflow=on  OutDataTypeStr=Inherit: Same as input  ParamDataTypeStr=Inherit: Same as input
  Quantizer : Quantizer  QuantizationInterval=param.meas.adc_quantization
  out : Outport
  wires:
  in/1 -> 1/Ti3/1
  1/Ti3/1 -> Quantizer/1
  Quantizer/1 -> out/1

== system single_phase_afe_ttype/single_phase_inverter/single phase inverter control/acquisition_and_scaling_grid_voltage_ac ==
  in : Inport
  1/Ti5 : Gain  Gain=1/param.grid.emu.u2bez  SaturateOnIntegerOverflow=on  OutDataTypeStr=Inherit: Same as input  ParamDataTypeStr=Inherit: Same as input
  Quantizer : Quantizer  QuantizationInterval=param.meas.adc_quantization
  out : Outport
  wires:
  Quantizer/1 -> out/1
  1/Ti5/1 -> Quantizer/1
  in/1 -> 1/Ti5/1

== system single_phase_afe_ttype/single_phase_inverter/single phase inverter control/acquisition_and_scaling_voltage ==
  in : Inport
  1/Ti5 : Gain  Gain=1/param.afe.hw.ubez  SaturateOnIntegerOverflow=on  OutDataTypeStr=Inherit: Same as input  ParamDataTypeStr=Inherit: Same as input
  Quantizer : Quantizer  QuantizationInterval=param.meas.adc_quantization
  pwm filtering for measure : cstblocks_lti/LTI System  sys=param.afe.ctrl.sogi.flt_beta  IC=[]  PadeOrder=0
  out : Outport
  wires:
  in/1 -> 1/Ti5/1
  pwm filtering for measure/1 -> Quantizer/1
  1/Ti5/1 -> pwm filtering for measure/1
  Quantizer/1 -> out/1

== system single_phase_afe_ttype/single_phase_inverter/single phase inverter control/inverter_current_output_pu_reference ==
  Gain : Gain
  Rate Limiter : RateLimiter  RisingSlewLimit=param.afe.ref.slew  FallingSlewLimit=-param.afe.ref.slew  SampleTimeMode=inherited
  Sum : Sum  Inputs=+++
  i_out_inverter_reference_step1 : Step  Time=param.afe.ref.t_1  FinalValue=param.afe.ref.i_pu_1  SampleTime=0
  i_out_inverter_reference_step2 : Step  Time=param.afe.ref.t_2  FinalValue=param.afe.ref.i_pu_2  SampleTime=0
  i_out_inverter_reference_step3 : Step  Time=param.afe.ref.t_3  FinalValue=param.afe.ref.i_pu_3  SampleTime=0
  inverter_current_output_pu_reference : Outport
  wires:
  Rate Limiter/1 -> Gain/1
  Sum/1 -> Rate Limiter/1
  Gain/1 -> inverter_current_output_pu_reference/1
  i_out_inverter_reference_step1/1 -> Sum/2
  i_out_inverter_reference_step2/1 -> Sum/3
  i_out_inverter_reference_step3/1 -> Sum/1
